simulink model "tcp_ip"  (R2021b)
settings: Solver=ode5  StartTime=0.0  StopTime=inf  FixedStep=1/20  RelTol=1e-3
PreLoadFcn:
  | mbxruntime.callbacks.PreLoadFcn(bdroot);
PostLoadFcn:
  | mbxruntime.callbacks.PostLoadFcn(bdroot);
InitFcn:
  | mbxruntime.callbacks.InitFcn(bdroot);
StartFcn:
  | mbxruntime.callbacks.StartFcn(bdroot);
StopFcn:
  | mbxruntime.callbacks.StopFcn(bdroot);
model workspace: external: MAT-File .\kea_demo_0218_cs_hws.mat (data not in the file)
undefined symbols (not defined in the file): DiscIntNeverNeededParam, kea_demo_0218_cs_1d5c9b61e8e009e5, kea_demo_0218_cs_4669f259e7287783, kea_demo_0218_cs_87ee11d7829c0052, kea_demo_0218_cs_Audi_A3_1_Dynamics_Simple_initialPitch, kea_demo_0218_cs_Audi_A3_1_Dynamics_Simple_initialRoll, kea_demo_0218_cs_Audi_A3_1_Dynamics_Simple_initialX, kea_demo_0218_cs_Audi_A3_1_Dynamics_Simple_initialY, kea_demo_0218_cs_Audi_A3_1_Dynamics_Simple_initialYaw, kea_demo_0218_cs_Audi_A3_1_Dynamics_Simple_initialZ, kea_demo_0218_cs_Audi_A3_1_PathFollower_Preview_1_PathUniqueID, kea_demo_0218_cs_Roewe_550_S_Sedan_1_Dynamics_Simple_initialX, kea_demo_0218_cs_Roewe_550_S_Sedan_1_Dynamics_Simple_initialY, kea_demo_0218_cs_Roewe_550_S_Sedan_1_Dynamics_Simple_initialYaw, kea_demo_0218_cs_Roewe_550_S_Sedan_1_Dynamics_Simple_initialZ, mbxruntime, warningInitialVelocity, x0
libraries: simulink x56, simulink_extras x18, instrumentlib x2
(part 4 of 7)

== system tcp_ip/Audi_A3_1/Dynamics_Simple/State2Bus1/state2FullState ==
  note: wrt GLOB
  note: Angles
      | wrtINI
  note: mode: Positioning
      | VelVEHICLE
      | wrt INI
  note: mode: Dynamics
      | VelVEHICLE
      | wrt VEH
  note: AnglesBODY
      | wrt GLOB
  note: AnglesVEHICLE
      | wrtGLOB
  note: AnglesBODY
      | wrtVEH
  dx,dy,dz [m/s] R,P,Y [rad] : Inport
  ini VEHpos wrt GLOB axis system [m] : Inport  Port=2
  iniBODY Angles wrt VEH axis system [deg] : Inport  Port=3
  iniVEH Angles wrt GLOB axis system [deg] : Inport  Port=4
  Degrees to Radians : simulink_extras/Transformations/Degrees to Radians
  Degrees to Radians1 : simulink_extras/Transformations/Degrees to Radians
  Demux : Demux  Outputs=3
  Demux1 : Demux  Outputs=[3 3 3]
  Demux2 : Demux  Outputs=[2 1]
  Demux3 : Demux  Outputs=2
  Demux4 : Demux  Outputs=3
  Discrete Derivative : simulink/Discrete/Discrete Derivative  gainval=1.0  ICPrevScaledInput=0.0  OutMin=[]  OutMax=[]  OutDataType=fixdt(1, 16)  OutScaling=2^-10  DoSatur=off
  Discrete Derivative1 : simulink/Discrete/Discrete Derivative  gainval=1.0  ICPrevScaledInput=0.0  OutMin=[]  OutMax=[]  OutDataType=fixdt(1, 16)  OutScaling=2^-10  DoSatur=off
  Discrete Derivative2 : simulink/Discrete/Discrete Derivative  gainval=1.0  ICPrevScaledInput=0.0  OutMin=[]  OutMax=[]  OutDataType=fixdt(1, 16)  OutScaling=2^-10  DoSatur=off
  Discrete Derivative3 : simulink/Discrete/Discrete Derivative  gainval=1.0  ICPrevScaledInput=str2num(get_param(gcb,'gainval'))*((Roll0*pi/180)/TimeStep)  OutMin=[]  OutMax=[]  OutDataType=fixdt(1, 16)  OutScaling=2^-10  DoSatur=off
  Discrete Derivative4 : simulink/Discrete/Discrete Derivative  gainval=1.0  ICPrevScaledInput=str2num(get_param(gcb,'gainval'))*((Pitch0*pi/180)/TimeStep)  OutMin=[]  OutMax=[]  OutDataType=fixdt(1, 16)  OutScaling=2^-10  DoSatur=off
  Discrete Derivative5 : simulink/Discrete/Discrete Derivative  gainval=1.0  ICPrevScaledInput=str2num(get_param(gcb,'gainval'))*((Yaw0*pi/180)/TimeStep)  OutMin=[]  OutMax=[]  OutDataType=fixdt(1, 16)  OutScaling=2^-10  DoSatur=off
  Mux : Mux  Inputs=[3 3 3 3 3]
  Mux1 : Mux  Inputs=3
  Mux2 : Mux  Inputs=3
  Sum : Sum  Inputs=|++
  Sum1 : Sum
  Sum2 : Sum
  Sum3 : Sum
  Transformation_BODY2GLOBAL : Subsystem
  Transformation_BODY2GLOBAL1 : Subsystem
  limit roll : Subsystem
  mux2 : Mux  Inputs=3
  mux3 : Mux  Inputs=3
  pitch_vehicle : Constant  Value=0
  roll_vehicle : Constant  Value=0
  yaw_body : Constant  Value=0
  State : Outport  VectorParamsAs1DForOutWhenUnconnected=off
  wires:
  Discrete Derivative5/1 -> Mux2/3
  Demux4/3 -> Discrete Derivative5/1
  Discrete Derivative4/1 -> Mux2/2
  Demux4/2 -> Discrete Derivative4/1
  Demux4/1 -> Discrete Derivative3/1
  Discrete Derivative3/1 -> Mux2/1
  Discrete Derivative2/1 -> Mux1/3
  Demux/3 -> Discrete Derivative2/1
  Discrete Derivative1/1 -> Mux1/2
  Demux/2 -> Discrete Derivative1/1
  Demux/1 -> Discrete Derivative/1
  Mux1/1 -> Mux/3  "AccVEH wrt  GLOB"
  Demux3/2 -> mux2/2  "pitch"
  ini VEHpos wrt GLOB axis system [m]/1 -> Sum3/2
  Degrees to Radians/1 -> Transformation_BODY2GLOBAL1/2(angles_BODYwrtGLOB_[rad]), Transformation_BODY2GLOBAL/2(angles_BODYwrtGLOB_[rad]), Sum2/2
  Degrees to Radians1/1 -> Sum1/2
  Demux3/1 -> mux2/1  "roll"
  Demux1/3 -> Demux2/1
  Demux2/1 -> Demux3/1
  Demux2/2 -> mux3/3  "yaw"
  Sum3/1 -> Mux/1  "PosVEH wrt  GLOB"
  Transformation_BODY2GLOBAL1/1(POSvector_GLOBAL_[m]) -> Sum3/1
  Sum1/1 -> Sum/1
  Demux1/1 -> Transformation_BODY2GLOBAL1/1(POSvector_BODY_[m])
  Transformation_BODY2GLOBAL/1(Vvector_GLOBAL_[m/s]) -> Demux/1, Mux/2  "VelVEH wrt  GLOB"
  dx,dy,dz [m/s] R,P,Y [rad]/1 -> Demux1/1
  Demux1/2 -> Transformation_BODY2GLOBAL/1(Vvector_BODY_[m/s])
  Sum2/1 -> Sum/2
  mux3/1 -> Sum2/1
  yaw_body/1 -> mux2/3  "yaw"
  mux2/1 -> Sum1/1
  pitch_vehicle/1 -> mux3/2  "pitch"
  roll_vehicle/1 -> mux3/1  "roll"
  Sum/1 -> limit roll/1(RPY)
  iniBODY Angles wrt VEH axis system [deg]/1 -> Degrees to Radians1/1
  iniVEH Angles wrt GLOB axis system [deg]/1 -> Degrees to Radians/1
  limit roll/1(RPYcor) -> Demux4/1, Mux/4  "AnglesBODY wrt  GLOB"
  Mux/1 -> State/1
  Mux2/1 -> Mux/5  "VelAnglesBODY wrt GLOB"
  Discrete Derivative/1 -> Mux1/1

== system tcp_ip/Audi_A3_1/Dynamics_Simple/Transmission/Torque_Converter ==
  note: <= 0
  note: > 0
  note: To compensate for no hydraulic connection when in neutral gear
  nEngine_[rpm] : Inport
  nTransmission_[rpm] : Inport  Port=2
  Gear nr : Inport  Port=3
  Compare To Constant : simulink/Logic and Bit Operations/Compare To Constant  relop=<=  const=1  OutDataTypeStr=uint8  ZeroCross=off
  Compare To Zero : simulink/Logic and Bit Operations/Compare To Zero  relop=~=  OutDataTypeStr=uint8  ZeroCross=off
  Constant : Constant  Value=1/50
  Constant1 : Constant
  Constant2 : Constant
  Drag : Gain  Gain=-1
  FactorK : Lookup  InputValues=p.speedratio  Table=p.Kfactor*p.Kcorr  SaturateOnIntegerOverflow=on
  Impeller : Fcn  Expr=u^2
  Product : Product  RndMeth=Zero
  Product1 : Product  RndMeth=Zero
  Quotient : Product  Inputs=*/  InputSameDT=on  SaturateOnIntegerOverflow=on  OutDataTypeStr=Inherit: Same as first input
  SpeedRatio : Product  Inputs=*/  InputSameDT=on  SaturateOnIntegerOverflow=on  OutDataTypeStr=Inherit: Same as first input
  Sum : Sum  Inputs=|+-
  Switch : Switch  Criteria=u2 ~= 0  Threshold=0.5
  Switch1 : Switch  Criteria=u2 ~= 0
  TorqueRatio : Lookup  InputValues=[p.speedratio 1]  Table=[p.Torqueratio 0]  SaturateOnIntegerOverflow=on
  Turbine : Product  InputSameDT=on  SaturateOnIntegerOverflow=on  OutDataTypeStr=Inherit: Same as first input
  rpm2rads-1 : Gain  Gain=2*pi/60
  ImpellerTorque_[Nm] : Outport  InitialOutput=0  VectorParamsAs1DForOutWhenUnconnected=off
  TurbineTorque_[Nm] : Outport  Port=2  InitialOutput=0  VectorParamsAs1DForOutWhenUnconnected=off
  wires:
  rpm2rads-1/1 -> Quotient/1
  Turbine/1 -> Switch1/1
  TorqueRatio/1 -> Turbine/2
  Compare To Constant/1 -> Switch1/2
  Constant2/1 -> Sum/2
  Sum/1 -> Drag/1
  Drag/1 -> Switch1/3
  Product1/1 -> TurbineTorque_[Nm]/1
  Switch1/1 -> Product1/2
  Compare To Zero/1 -> Switch/2
  Gear nr/1 -> Compare To Zero/1
  Constant1/1 -> Switch/1
  Constant/1 -> Switch/3
  Switch/1 -> Product1/1, Product/1
  Product/1 -> ImpellerTorque_[Nm]/1
  Quotient/1 -> Impeller/1
  FactorK/1 -> Quotient/2
  SpeedRatio/1 -> FactorK/1, Sum/1, Compare To Constant/1, TorqueRatio/1
  Impeller/1 -> Turbine/1, Product/2
  nEngine_[rpm]/1 -> SpeedRatio/2, rpm2rads-1/1
  nTransmission_[rpm]/1 -> SpeedRatio/1

== system tcp_ip/Audi_A3_1/Dynamics_Simple/Transmission/Transmission_Ratio ==
  tTransmissionIn_[Nm] : Inport
  GearNr_[-] : Inport  Port=2
  nTransmissionOut_[rpm] : Inport  Port=3
  Ensure positive TransmissionRPM : Abs
  If : If  IfExpression=u1 == 0  ElseIfExpressions=u1 == -1
  If Action Neutral : Subsystem  TreatAsAtomicUnit=on
  If Action Normal : Subsystem  TreatAsAtomicUnit=on
  If Action Reverse : Subsystem  TreatAsAtomicUnit=on
  Merge : Merge  Inputs=3
  OutputTorque = 0 : Constant  Value=0
  Product : Product  InputSameDT=on  SaturateOnIntegerOverflow=on  OutDataTypeStr=Inherit: Same as first input
  Product1 : Product  InputSameDT=on  SaturateOnIntegerOverflow=on  OutDataTypeStr=Inherit: Same as first input
  Transmission Gear ratios : Lookup  InputValues=p.tr_in  Table=p.tr_out  SaturateOnIntegerOverflow=on
  tTransmissionOut_[Nm] : Outport  InitialOutput=0  VectorParamsAs1DForOutWhenUnconnected=off
  nTransmissionIn_[rpm] : Outport  Port=2  InitialOutput=0  VectorParamsAs1DForOutWhenUnconnected=off
  wires:
  GearNr_[-]/1 -> Transmission Gear ratios/1, If/1
  If/3 -> If Action Normal/Action
  If/2 -> If Action Reverse/Action
  If Action Normal/1(Out1) -> Merge/3
  If Action Reverse/1(Out1) -> Merge/2
  If/1 -> If Action Neutral/Action
  If Action Neutral/1(Out1) -> Merge/1
  Product1/1 -> Ensure positive TransmissionRPM/1
  Merge/1 -> tTransmissionOut_[Nm]/1
  Product/1 -> If Action Reverse/1(In1), If Action Normal/1(In1)
  OutputTorque = 0/1 -> If Action Neutral/1(In1)
  Transmission Gear ratios/1 -> Product/2, Product1/1
  nTransmissionOut_[rpm]/1 -> Product1/2
  tTransmissionIn_[Nm]/1 -> Product/1
  Ensure positive TransmissionRPM/1 -> nTransmissionIn_[rpm]/1

== system tcp_ip/Audi_A3_1/PathFollower_Preview_1/LateralController/Calculate delta wheel ==
  In1 : Inport
  In2 : Inport  Port=2
  In3 : Inport  Port=3
  In4 : Inport  Port=4
  In5 : Inport  Port=5
  In6 : Inport  Port=6
  In7 : Inport  Port=7
  In8 : Inport  Port=8
  In9 : Inport  Port=9
  In10 : Inport  Port=10
  In11 : Inport  Port=11
  In12 : Inport  Port=12
  eml_delta_steering_error : MATLAB Function  TreatAsAtomicUnit=on  RTWFcnName=sfun_delta_steering_error  RTWFileName=sfun_delta_steering_error
      settings: RTWFileNameOpts=User specified
  Out1 : Outport  VectorParamsAs1DForOutWhenUnconnected=off
  wires:
  In3/1 -> eml_delta_steering_error/3(t_Preview_LatCtrl)
  In2/1 -> eml_delta_steering_error/2(v_x_vehicle_Min)
  In12/1 -> eml_delta_steering_error/12(wheelbase)
  In11/1 -> eml_delta_steering_error/11(Pos_x_CoG_Vehicle)
  In10/1 -> eml_delta_steering_error/10(e_Lat)
  In9/1 -> eml_delta_steering_error/9(inertia_z_vehicle_total)
  In8/1 -> eml_delta_steering_error/8(m_vehicle_total)
  eml_delta_steering_error/1(delta_steeringwheeltotal) -> Out1/1
  In7/1 -> eml_delta_steering_error/7(CorneringStiffness_Tyres_Rear)
  In6/1 -> eml_delta_steering_error/6(CorneringStiffness_Tyres_Front)
  In5/1 -> eml_delta_steering_error/5(yawrate_vehicle)
  In4/1 -> eml_delta_steering_error/4(v_y_vehicle)
  In1/1 -> eml_delta_steering_error/1(v_x_vehicle)

== system tcp_ip/Audi_A3_1/PathFollower_Preview_1/LateralController/SteeringWheelAngle ==
  Angle_Steering[rad] : Inport
  i_Steering[] : Inport  Port=2
  Angle_SteeringWheel_Last[deg] : Inport  Port=3
  LatCtrl1_Enable[0Off|1On] : Inport  Port=4
  Angle_Max_SteeringWheel[deg]1 : Constant  Value=Angle_Max_SteeringWheel  SampleTime=CSSampleTime
  Const_t_PT1_LatCtrl[s] : Constant  Value=DelayTime  SampleTime=CSSampleTime
  FirstOrderDynamics : Subsystem  mask(First Order Dynamics){}
      mask Display:
      | port_label('input',1,'In')
      | port_label('input',2,'T')
      | port_label('input',3,'Reset')
      | port_label('input',4,'x0')
      | 
      | plot([0.4 0.95], [0.1 0.1]);
      | plot([0.4 0.4], [0.1 0.95]);
      | plot(0.4 + 0.5*[0:0.1:1],0.8- 0.7 * exp(-5*[0:0.1:1]));
  Gain : Gain  SaturateOnIntegerOverflow=on  OutDataTypeStr=Inherit: Same as input  ParamDataTypeStr=Inherit: Same as input
  Product : Product  SaturateOnIntegerOverflow=on  OutDataTypeStr=Inherit: Same as first input
  Rate Limiter : RateLimiter  RisingSlewLimit=MaxSteeringRate  FallingSlewLimit=-MaxSteeringRate  SampleTimeMode=inherited
  Sat_Total : Subsystem
      mask Display:
      | plot([0.25 0.4 0.6 0.75],[0.2 0.2 0.8 0.8])
      | port_label('input',2,'Lim')
      | port_label('output',2,'Info')
  Terminator1 : Terminator
  rad2deg : Gain  Gain=180/pi  SaturateOnIntegerOverflow=on  OutDataTypeStr=Inherit: Same as input  ParamDataTypeStr=Inherit: Same as input
  Angle_SteeringWheel[deg] : Outport  VectorParamsAs1DForOutWhenUnconnected=off
  wires:
  Rate Limiter/1 -> FirstOrderDynamics/1(In)
  Gain/1 -> FirstOrderDynamics/3(Reset)
  Angle_SteeringWheel_Last[deg]/1 -> FirstOrderDynamics/4(x0)
  LatCtrl1_Enable[0Off|1On]/1 -> Gain/1
  Const_t_PT1_LatCtrl[s]/1 -> FirstOrderDynamics/2(TimeConstant[s])
  Sat_Total/2(Sat_Info) -> Terminator1/1
  Angle_Steering[rad]/1 -> rad2deg/1
  i_Steering[]/1 -> Product/2
  rad2deg/1 -> Product/1
  Product/1 -> Sat_Total/1(In)
  Sat_Total/1(Sat_Total) -> Rate Limiter/1
  FirstOrderDynamics/1(Out) -> Angle_SteeringWheel[deg]/1
  Angle_Max_SteeringWheel[deg]1/1 -> Sat_Total/2(Sat_Limit)

== system tcp_ip/Audi_A3_1/PathFollower_Preview_1/LateralController/s_Preview_LatCtrl ==
  v_x_Vehicle[m|s] : Inport
  v_x_Vehicle_Min[m|s] : Inport  Port=2
  t_Preview_LatCtrl[s] : Inport  Port=3
  Max : MinMax  Function=max  Inputs=2  InputSameDT=on  SaturateOnIntegerOverflow=on
  Prod_s_Min : Product  SaturateOnIntegerOverflow=on  OutDataTypeStr=Inherit: Same as first input
  Product : Product  SaturateOnIntegerOverflow=on  OutDataTypeStr=Inherit: Same as first input
  s_Preview_LatCtrl[m] : Outport  VectorParamsAs1DForOutWhenUnconnected=off
  wires:
  Max/1 -> s_Preview_LatCtrl[m]/1
  Prod_s_Min/1 -> Max/2
  v_x_Vehicle_Min[m|s]/1 -> Prod_s_Min/2
  t_Preview_LatCtrl[s]/1 -> Prod_s_Min/1, Product/2
  Product/1 -> Max/1
  v_x_Vehicle[m|s]/1 -> Product/1

== system tcp_ip/Audi_A3_1/PathFollower_Preview_1/LongitudinalController/Check_Initial_Velocity ==
  " v_actual_[m|s]" : Inport
  Initial_Velocity_[m|s] : Inport  Port=2
  > eps : simulink/Logic and Bit Operations/Compare To Constant  relop=>  const=0.1  OutDataTypeStr=boolean
  Abs : Abs
  Assertion : Assertion  AssertionFailFcn=warningInitialVelocity(PathFollowerBlockPath);  StopWhenAssertionFail=off
  Constant : Constant  Value=false
  First ? : Memory  InitialCondition=1
  Logical Operator : Logic  AllPortsSameDT=off  OutDataTypeStr=boolean
  Logical Operator1 : Logic  Operator=NOT  AllPortsSameDT=off  OutDataTypeStr=boolean
  Sum : Sum  Inputs=+-
  wires:
  Logical Operator1/1 -> Assertion/1
  Logical Operator/1 -> Logical Operator1/1
  Constant/1 -> First ?/1
  First ?/1 -> Logical Operator/2
  > eps/1 -> Logical Operator/1
  Sum/1 -> Abs/1
  Abs/1 -> > eps/1
  Initial_Velocity_[m|s]/1 -> Sum/2
  " v_actual_[m|s]"/1 -> Sum/1

== system tcp_ip/Audi_A3_1/PathFollower_Preview_1/LongitudinalController/If Desired Velocity = 0 ==
  In1 : Inport
  Action Port : ActionPort  InitializeStates=reset  PropagateVarSize=During execution  ActionPortLabel=if(u1 == 0)
  constant : Constant  Value=0
  constant1 : Constant  Value=150
  throttle [%] : Outport  InitialOutput=[0]  VectorParamsAs1DForOutWhenUnconnected=off
  brake pressure [bar] : Outport  Port=2  InitialOutput=[150]  VectorParamsAs1DForOutWhenUnconnected=off
  Auto_GearShift : Outport  Port=3  VectorParamsAs1DForOutWhenUnconnected=off
  wires:
  In1/1 -> Auto_GearShift/1
  constant/1 -> throttle [%]/1
  constant1/1 -> brake pressure [bar]/1

== system tcp_ip/Audi_A3_1/PathFollower_Preview_1/LongitudinalController/If Desired Velocity ~= 0 ==
  note: No brake/throttle actions
      | in case of small ctrl error,
      |  in order to prevent nervous
      | ctrl behaviour
  note: CONSTANT VELOCITY CONTROL
  In1 : Inport
  Desired Velocity [m/s] : Inport  Port=2
  Action Port : ActionPort  InitializeStates=reset  PropagateVarSize=During execution  ActionPortLabel=else
  Dead Zone1 : DeadZone  LowerValue=-10  UpperValue=1  SaturateOnIntegerOverflow=on
  Gain1 : Gain  Gain=-1
  Gain2 : Gain  Gain=1.5
  Limiter_brake : Saturate  UpperLimit=150  LowerLimit=0
  Limiter_throttle : Saturate  UpperLimit=100  LowerLimit=0
  PID_AWU : Subsystem  mask(PID Controller){P=LongCtrl_P, I=LongCtrl_I, D=LongCtrl_D}
      mask prompts: P "Proportional:"; I "Integral:"; D "Derivative:"
      mask help:
      | Enter expressions for proportional, integral, and derivative terms.
      | P+I/s+Ds
      mask Help: This block implements a PID controller where parameters are entered for the Proportional, Integral and Derivative terms. Unmask this block to see how it works. The derivative term is implemented using a true derivative block.
      mask Display: disp('PID')
  throttle [%] : Outport  VectorParamsAs1DForOutWhenUnconnected=off
  brake pressure [bar] : Outport  Port=2  VectorParamsAs1DForOutWhenUnconnected=off
  Auto_GearShift : Outport  Port=3  VectorParamsAs1DForOutWhenUnconnected=off
  wires:
  Dead Zone1/1 -> Gain2/1, Limiter_throttle/1
  Gain1/1 -> Limiter_brake/1
  Gain2/1 -> Gain1/1
  PID_AWU/1(u) -> Dead Zone1/1
  Desired Velocity [m/s]/1 -> PID_AWU/1(e)
  In1/1 -> Auto_GearShift/1
  Limiter_brake/1 -> brake pressure [bar]/1
  Limiter_throttle/1 -> throttle [%]/1  "throttle"

== system tcp_ip/Audi_A3_1/PathFollower_Preview_1/LongitudinalController/Memory External IC ==
  note: Xnew
  note: Initial Value
  u : Inport
  IC : Inport  Port=2
  FixPt Constant : Constant  DisableCoverage=on  Value=0  OutDataTypeStr=fixdt(0,8,0)
  FixPt Data Type Duplicate1 : DataTypeDuplicate  DisableCoverage=on  NumInputPorts=3
  Init : Switch  Criteria=u2 ~= 0  OutDataTypeStr=Inherit: Inherit via back propagation  ZeroCross=off
  Memory : Memory  InitialCondition=1  InheritSampleTime=on
  Memory1 : Memory  InheritSampleTime=on
  y : Outport  VectorParamsAs1DForOutWhenUnconnected=off
  wires:
  Memory1/1 -> Init/3  "Xold"
  Init/1 -> y/1, FixPt Data Type Duplicate1/1
  Memory/1 -> Init/2
  FixPt Constant/1 -> Memory/1
  u/1 -> Memory1/1, FixPt Data Type Duplicate1/2
  IC/1 -> Init/1, FixPt Data Type Duplicate1/3

== system tcp_ip/Audi_A3_1/SELF_Demux/compas converter/cart2compas ==
  Angle [deg] : Inport
  Constant : Constant  Value=90
  Constant1 : Constant  Value=360
  Gain : Gain  Gain=1/360
  Gain1 : Gain  Gain=360
  Gain2 : Gain  Gain=-1
  Rounding Function : Rounding
  Sum : Sum  Inputs=|-+
  Sum1 : Sum  Inputs=-+|
  Sum2 : Sum  Inputs=++|
  heading [deg] : Outport  VectorParamsAs1DForOutWhenUnconnected=off
  wires:
  Gain/1 -> Rounding Function/1
  Rounding Function/1 -> Gain1/1
  Gain1/1 -> Sum/1
  Angle [deg]/1 -> Sum1/2
  Sum/1 -> Gain2/1
  Sum1/1 -> Gain/1, Sum/2
  Constant/1 -> Sum1/1
  Gain2/1 -> Sum2/2
  Constant1/1 -> Sum2/1
  Sum2/1 -> heading [deg]/1

== system tcp_ip/Roewe_550_S_Sedan_1/Dynamics_Simple/Chassis/Bicycle_model_[XYZ] ==
  DeltaWheel_[rad] : Inport
  zFront_[m]_dzFront_[ms-1] : Inport  Port=2  PortDimensions=2
  zRear_[m]_dzRear_[ms-1] : Inport  Port=3  PortDimensions=2
  BrakePressure_[bar] : Inport  Port=4
  DriveTorque_[Nm] : Inport  Port=5
  v0_[ms-1] : Inport  Port=6
  |vx|_[ms-1] : Inport  Port=7
  Fy_rear_[N] : Inport  Port=8
  Fy_front_[N] : Inport  Port=9
  Demux : Demux  Outputs=2
  Demux1 : Demux  Outputs=2
  Fyi --> Fy / Mz : Subsystem
  X_Motion : Subsystem
  Y & Yaw_Motion : Subsystem
  "Z, Pitch_Motion & Roll_Motion" : Subsystem
  |vx|_[ms-1]1 : Outport  VectorParamsAs1DForOutWhenUnconnected=off
  vy_[ms-1] : Outport  Port=2  VectorParamsAs1DForOutWhenUnconnected=off
  vz_[ms-1] : Outport  Port=3  VectorParamsAs1DForOutWhenUnconnected=off
  RollAngle_[rad] : Outport  Port=4  VectorParamsAs1DForOutWhenUnconnected=off
  RollRate_[rads-1] : Outport  Port=5  VectorParamsAs1DForOutWhenUnconnected=off
  YawAngle_[rads-1] : Outport  Port=6  VectorParamsAs1DForOutWhenUnconnected=off
  Vx_[ms-1] : Outport  Port=7  VectorParamsAs1DForOutWhenUnconnected=off
  PitchAngle_[rad] : Outport  Port=8  VectorParamsAs1DForOutWhenUnconnected=off
  YawAngle_[rad] : Outport  Port=9  VectorParamsAs1DForOutWhenUnconnected=off
  ax_[ms-2] : Outport  Port=10  VectorParamsAs1DForOutWhenUnconnected=off
  ay_[ms-2] : Outport  Port=11  VectorParamsAs1DForOutWhenUnconnected=off
  wires:
  Fyi --> Fy / Mz/1(Fy_[N]) -> Y & Yaw_Motion/2(Fy_[N])  "Fy_[N]"
  Fyi --> Fy / Mz/2(Mz_[Nm]) -> Y & Yaw_Motion/3(Mz_[Nm])  "Mz_[Nm]"
  Y & Yaw_Motion/1(|vx|_[ms-1]1) -> |vx|_[ms-1]1/1  "|vx|_[ms-1]"
  Y & Yaw_Motion/2(vy_[ms-1]) -> vy_[ms-1]/1  "vy_[ms-1]"
  Y & Yaw_Motion/5(YawAngle_[rad]) -> YawAngle_[rad]/1  "YawAngle_[rad]"
  v0_[ms-1]/1 -> X_Motion/3(v0_[ms-1])  "v0_[ms-1]"
  BrakePressure_[bar]/1 -> X_Motion/2(BrakePressure_[bar])  "BrakePressure_[bar]"
  DriveTorque_[Nm]/1 -> X_Motion/1(DriveTorque_[Nm])  "DriveTorque_[Nm]"
  X_Motion/2(ax_[ms-2]) -> ax_[ms-2]/1, [ax]  "ax_[ms-2]"
  X_Motion/1(vx_[ms-1]) -> Vx_[ms-1]/1, [vx]  "vx_[ms-1]"
  [ax] -> "Z, Pitch_Motion & Roll_Motion"/3(ax)
  Demux/1 -> "Z, Pitch_Motion & Roll_Motion"/5(zFront_[m])
  Demux/2 -> "Z, Pitch_Motion & Roll_Motion"/6(dzFront_[ms-1])
  Demux1/1 -> "Z, Pitch_Motion & Roll_Motion"/7(zRear_[m])
  Demux1/2 -> "Z, Pitch_Motion & Roll_Motion"/8(dzRear_[ms-1])
  zRear_[m]_dzRear_[ms-1]/1 -> Demux1/1
  zFront_[m]_dzFront_[ms-1]/1 -> Demux/1
  "Z, Pitch_Motion & Roll_Motion"/2(vz_[ms-1]) -> vz_[ms-1]/1  "vz_[ms-1]"
  DeltaWheel_[rad]/1 -> Fyi --> Fy / Mz/1(DeltaWheel_[rad])
  Fy_front_[N]/1 -> Fyi --> Fy / Mz/2(Fy_f_[N])
  Fy_rear_[N]/1 -> Fyi --> Fy / Mz/3(Fy_r_[N])
  |vx|_[ms-1]/1 -> Y & Yaw_Motion/1(|vx|_[ms-1])
  Y & Yaw_Motion/3(ay_[ms-2]) -> [ay], ay_[ms-2]/1  "ay_[ms-2]"
  [ay] -> "Z, Pitch_Motion & Roll_Motion"/4(ay)
  "Z, Pitch_Motion & Roll_Motion"/3(RollAngle_[rad]) -> RollAngle_[rad]/1  "RollAngle_[rad]"
  "Z, Pitch_Motion & Roll_Motion"/4(RollRate_[rads-1]) -> RollRate_[rads-1]/1  "RollRate_[rads-1]"
  [dYaw] -> "Z, Pitch_Motion & Roll_Motion"/2(dYaw)
  [vx] -> "Z, Pitch_Motion & Roll_Motion"/1(vx)
  Y & Yaw_Motion/4(dYawAngle_[rads-1]) -> YawAngle_[rads-1]/1, [dYaw]  "dYawAngle_[rads-1]"
  "Z, Pitch_Motion & Roll_Motion"/1(pitchAngle_[rad]) -> PitchAngle_[rad]/1  "PitchAngle_[rad]"

== system tcp_ip/Roewe_550_S_Sedan_1/Dynamics_Simple/Chassis/FrontTyre ==
  note: alpha limiter
      | [-1 ... 1]
  note: relax_on
      | ON: 1
      | OFF: 0
  note: MOTORCYCLE ONLY
  note: VEHICLE + MOTORCYCLE
  DeltaWheel_[rad] : Inport
  |vx|_[ms-1] : Inport  Port=2
  vy_[ms-1] : Inport  Port=3
  dYawAngle_[rads-1] : Inport  Port=4
  RollAngle_[rad] : Inport  Port=5
  AlphaFront : Subsystem
  Compare To Zero : simulink/Logic and Bit Operations/Compare To Zero  relop===  OutDataTypeStr=boolean  ZeroCross=off
  Configurable Subsystem : Subsystem  Variant=on  VariantControlMode=label  LabelModeActiveChoice=Continuous
      settings: AttributesFormatString=%<BlockChoice>  OpenFcn=BringToFront(gcb);
  Configurable Subsystem1 : Subsystem  Variant=on  VariantControlMode=label  LabelModeActiveChoice=Continuous
      settings: AttributesFormatString=%<BlockChoice>  OpenFcn=BringToFront(gcb);
  Constant : Constant  Value=p.relax_on
  Constant1 : Constant  Value=p.relax_on
  Constant2 : Constant  Value=p.VehMCSwitch
  Data Type Conversion : DataTypeConversion  OutDataTypeStr=double
  If MC : simulink/Logic and Bit Operations/Compare To Constant  relop===  const=2  OutDataTypeStr=uint8  ZeroCross=off
  K_gamma_front : Gain  Gain=p.Kgfront
  Linl : Fcn  Expr=(u(4) - u(5))/p.sigma_front*u(1)
  Linl1 : Fcn  Expr=(u(4) - u(5))/p.sigma_front*u(1)
  Mux1 : Mux  Inputs=3
  Mux2 : Mux  Inputs={3,1,1}
  Mux3 : Mux  Inputs={3,1,1}
  Prevent_instability_at_low_Vx : Subsystem
  Product : Product  RndMeth=Zero
  Sum : Sum  Inputs=|++  InputSameDT=on  SaturateOnIntegerOverflow=on  OutDataTypeStr=Inherit: Same as first input
  Sum1 : Sum  Inputs=|++
  Switch : Switch  Threshold=0.5  SaturateOnIntegerOverflow=on  InputSameDT=on
  Switch1 : Switch  Threshold=0.5  SaturateOnIntegerOverflow=on  InputSameDT=on
  alg.loop : Memory
  due to sign convention : Gain  Gain=-1  SaturateOnIntegerOverflow=on  OutDataTypeStr=Inherit: Same as input  ParamDataTypeStr=Inherit: Same as input
  front_tyre : Gain  Gain=p.Kfront
  FyFront_[N] : Outport  VectorParamsAs1DForOutWhenUnconnected=off
  wires:
  Prevent_instability_at_low_Vx/1(alpha [rad]) -> Mux2/2, Switch/3
  Sum/1 -> Prevent_instability_at_low_Vx/1(alpha[rad])  "AlphaStatFront_[rad]"
  Switch/1 -> front_tyre/1  "AlphaFront_[rad]"
  Constant/1 -> Switch/2
  Sum1/1 -> FyFront_[N]/1  "FyFront_[N]"
  Mux2/1 -> Linl/1
  Linl/1 -> Configurable Subsystem/1(In1)
  Configurable Subsystem/1(Out1) -> Mux2/3, Switch/1  "AlphaRelaxFront_[rad]"
  AlphaFront/1(Alpha) -> Sum/1
  Mux1/1 -> Prevent_instability_at_low_Vx/2(In), AlphaFront/1(In), Mux2/1, Mux3/1
  |vx|_[ms-1]/1 -> Mux1/1, Compare To Zero/1
  vy_[ms-1]/1 -> Mux1/2
  dYawAngle_[rads-1]/1 -> Mux1/3
  alg.loop/1 -> Switch1/3
  Configurable Subsystem1/1(Out1) -> Mux3/3, Switch1/1  "GammaRelaxFront_[rad]"
  Linl1/1 -> Configurable Subsystem1/1(In1)
  Mux3/1 -> Linl1/1
  Constant1/1 -> Switch1/2
  due to sign convention/1 -> alg.loop/1, Mux3/2  "GammaStatFront_[rad]"
  RollAngle_[rad]/1 -> due to sign convention/1
  front_tyre/1 -> Sum1/1
  Constant2/1 -> If MC/1
  If MC/1 -> Data Type Conversion/1
  K_gamma_front/1 -> Product/1
  Product/1 -> Sum1/2
  Data Type Conversion/1 -> Product/2
  Compare To Zero/1 -> [reset]
  [reset] -> Configurable Subsystem/2(In2)
  [reset] -> Configurable Subsystem1/2(In2)
  DeltaWheel_[rad]/1 -> Sum/2  "DeltaWheel_[rad]"
  Switch1/1 -> K_gamma_front/1  "GammaFront_[rad]"

== system tcp_ip/Roewe_550_S_Sedan_1/Dynamics_Simple/Chassis/MuxDynState ==
  note: The position inputs are computed by the
      | integrated velocity.
  note: mode: Dynamics
      | VelVEHICLE
      | wrt VEH
  note: AnglesVEHICLE
      | wrtGLOB
  vx [ms-1] : Inport
  vy [ms-1] : Inport  Port=2
  vz [ms-1] : Inport  Port=3
  R [rad] : Inport  Port=4
  P [rad] : Inport  Port=5
  Y [rad] : Inport  Port=6
  Configurable Subsystem1 : Subsystem  Variant=on  VariantControlMode=label  LabelModeActiveChoice=Continuous  mask{IntegrationMethod=Integrator: Forward Euler}
      mask prompts: IntegrationMethod "Integration method"
      mask init: same as tcp_ip/Audi_A3_1/Dynamics_Simple/Chassis/MuxDynState/Configurable Subsystem1
      settings: AttributesFormatString=%<BlockChoice>  OpenFcn=BringToFront(gcb);
      mask TypeOptions IntegrationMethod: Integrator: Forward Euler | Integrator: Backward Euler
  Ground : Ground
  Ground1 : Ground
  Mux : Mux  Inputs=[3 3 3]
  Mux1 : Mux  Inputs=3
  Mux2 : Mux  Inputs=3
  Transformation_BODY2GLOBAL : Subsystem
  mux3 : Mux  Inputs=3
  State : Outport  VectorParamsAs1DForOutWhenUnconnected=off
  wires:
  Ground1/1 -> mux3/2  "pitch"
  Y [rad]/1 -> Mux2/3, mux3/3  "yaw"
  P [rad]/1 -> Mux2/2
  R [rad]/1 -> Mux2/1
  vz [ms-1]/1 -> Mux1/3
  vy [ms-1]/1 -> Mux1/2
  vx [ms-1]/1 -> Mux1/1
  Mux2/1 -> Mux/3
  Transformation_BODY2GLOBAL/1(Vvector_GLOBAL_[m/s]) -> Configurable Subsystem1/1(In1), Mux/2  "VelVEH wrt  GLOB"
  mux3/1 -> Transformation_BODY2GLOBAL/2(angles_BODYwrtGLOB_[rad])
  Ground/1 -> mux3/1  "roll"
  Mux/1 -> State/1
  Mux1/1 -> Transformation_BODY2GLOBAL/1(Vvector_BODY_[m/s])
  Configurable Subsystem1/1(Out1) -> Mux/1  "PosVEH wrt  GLOB"

== system tcp_ip/Roewe_550_S_Sedan_1/Dynamics_Simple/Chassis/Power Assisted Steering ==
  note: MOTORCYCLE
  note: VEHICLE
  note: Reverse steering direction for negative velocities
  Vx_[ms-1] : Inport
  Delta_in_[deg] : Inport  Port=2
  Constant : Constant
  Constant1 : Constant  Value=p.VehMCSwitch
  Lookup Table : Lookup  InputValues=[0 35 45 100]  Table=[1 1 0.2 0.2]
  Multiport Switch : MultiPortSwitch  Inputs=2
  Product : Product  Inputs=3  RndMeth=Zero
  Sign : Signum
  Delta_out_[deg] : Outport  VectorParamsAs1DForOutWhenUnconnected=off
  wires:
  Vx_[ms-1]/1 -> Lookup Table/1, Sign/1
  Delta_in_[deg]/1 -> Product/3
  Constant1/1 -> Multiport Switch/1
  Constant/1 -> Multiport Switch/3
  Lookup Table/1 -> Multiport Switch/2
  Multiport Switch/1 -> Product/2
  Product/1 -> Delta_out_[deg]/1
  Sign/1 -> Product/1

== system tcp_ip/Roewe_550_S_Sedan_1/Dynamics_Simple/Chassis/RearTyre ==
  note: alpha limiter
      | [-1 ... 1]
  note: relax_on
      | ON: 1
      | OFF: 0
  note: MOTORCYCLE ONLY
  note: VEHICLE + MOTORCYCLE
  |vx|_[ms-1] : Inport
  vy_[ms-1] : Inport  Port=2
  dpsi_[rads-1] : Inport  Port=3
  RollAngle_[rad] : Inport  Port=4
  AlphaRear : Subsystem
  Compare To Zero : simulink/Logic and Bit Operations/Compare To Zero  relop===  OutDataTypeStr=boolean  ZeroCross=off
  Configurable Subsystem : Subsystem  Variant=on  VariantControlMode=label  LabelModeActiveChoice=Continuous
      settings: AttributesFormatString=%<BlockChoice>  OpenFcn=BringToFront(gcb);
  Configurable Subsystem1 : Subsystem  Variant=on  VariantControlMode=label  LabelModeActiveChoice=Continuous
      settings: AttributesFormatString=%<BlockChoice>  OpenFcn=BringToFront(gcb);
  Constant1 : Constant  Value=p.relax_on
  Constant2 : Constant  Value=p.relax_on
  Constant3 : Constant  Value=p.VehMCSwitch
  Data Type Conversion : DataTypeConversion  OutDataTypeStr=double
  If MC : simulink/Logic and Bit Operations/Compare To Constant  relop===  const=2  OutDataTypeStr=uint8  ZeroCross=off
  K_gamma_rear : Gain  Gain=p.Kgrear
  Linl : Fcn  Expr=(u(4) - u(5))/p.sigma_rear*u(1)
  Linl1 : Fcn  Expr=(u(4) - u(5))/p.sigma_rear*u(1)
  Mux1 : Mux  Inputs=3
  Mux2 : Mux  Inputs={3,1,1}
  Mux3 : Mux  Inputs={3,1,1}
  Prevent_instability_at_low_Vx : Subsystem
  Product : Product  RndMeth=Zero
  Sum1 : Sum  Inputs=|++
  Switch1 : Switch  Threshold=0.5  SaturateOnIntegerOverflow=on  InputSameDT=on
  Switch2 : Switch  Threshold=0.5  SaturateOnIntegerOverflow=on  InputSameDT=on
  alg.loop : Memory
  due to sign convention : Gain  Gain=-1  SaturateOnIntegerOverflow=on  OutDataTypeStr=Inherit: Same as input  ParamDataTypeStr=Inherit: Same as input
  rear_tyre : Gain  Gain=p.Krear
  FyRear_[N] : Outport  VectorParamsAs1DForOutWhenUnconnected=off
  wires:
  Prevent_instability_at_low_Vx/1(alpha [rad]) -> Switch1/3, Mux2/2
  AlphaRear/1(Alpha) -> Prevent_instability_at_low_Vx/1(alpha[rad])  "AlphaStatRear_[rad]"
  Switch1/1 -> rear_tyre/1  "AlphaRear_[rad]"
  Constant1/1 -> Switch1/2
  Sum1/1 -> FyRear_[N]/1  "FyRear_[N]"
  Mux2/1 -> Linl/1
  Linl/1 -> Configurable Subsystem1/1(In1)
  Configurable Subsystem1/1(Out1) -> Mux2/3, Switch1/1  "AlphaRelaxRear_[rad]"
  Mux1/1 -> Prevent_instability_at_low_Vx/2(In), AlphaRear/1(In), Mux2/1, Mux3/1
  |vx|_[ms-1]/1 -> Mux1/1, Compare To Zero/1
  vy_[ms-1]/1 -> Mux1/2
  dpsi_[rads-1]/1 -> Mux1/3
  alg.loop/1 -> Switch2/3
  Configurable Subsystem/1(Out1) -> Mux3/3, Switch2/1  "GammaRelaxRear_[rad]"
  Linl1/1 -> Configurable Subsystem/1(In1)
  Mux3/1 -> Linl1/1
  Constant2/1 -> Switch2/2
  due to sign convention/1 -> alg.loop/1, Mux3/2  "GammaStatRear_[rad]"
  RollAngle_[rad]/1 -> due to sign convention/1
  Constant3/1 -> If MC/1
  If MC/1 -> Data Type Conversion/1
  Product/1 -> Sum1/2
  Data Type Conversion/1 -> Product/2
  K_gamma_rear/1 -> Product/1
  rear_tyre/1 -> Sum1/1
  Compare To Zero/1 -> [reset]
  [reset] -> Configurable Subsystem1/2(In2)
  [reset] -> Configurable Subsystem/2(In2)
  Switch2/1 -> K_gamma_rear/1  "GammaFront_[rad]"

== system tcp_ip/Roewe_550_S_Sedan_1/Dynamics_Simple/Engine/Configurable Subsystem ==
  In1 : Inport
  Discrete Rate Limiter : Subsystem  VariantControl=Discrete
  Rate Limiter : Subsystem  VariantControl=Continuous
  Out1 : Outport  VectorParamsAs1DForOutWhenUnconnected=off

== system tcp_ip/Roewe_550_S_Sedan_1/Dynamics_Simple/Engine/Configurable Subsystem1 ==
  In1 : Inport
  Discrete-Time Integrator : Subsystem  VariantControl=Discrete
  Integrator : Subsystem  VariantControl=Continuous
  Out1 : Outport  VectorParamsAs1DForOutWhenUnconnected=off

== system tcp_ip/Roewe_550_S_Sedan_1/Dynamics_Simple/Gear: Auto Manual/If Action Subsystem ==
  In1 : Inport
  Action Port : ActionPort  PropagateVarSize=During execution  ActionPortLabel=if(u1 == 0)
  Out1 : Outport  VectorParamsAs1DForOutWhenUnconnected=off
  wires:
  In1/1 -> Out1/1

== system tcp_ip/Roewe_550_S_Sedan_1/Dynamics_Simple/Gear: Auto Manual/If Action Subsystem1 ==
  In1 : Inport
  Action Port : ActionPort  PropagateVarSize=During execution  ActionPortLabel=else
  Out1 : Outport  VectorParamsAs1DForOutWhenUnconnected=off
  wires:
  In1/1 -> Out1/1

== system tcp_ip/Roewe_550_S_Sedan_1/Dynamics_Simple/ShiftLogic/Detect Increase ==
  GearNr_[-] : Inport
  In2 : Inport  Port=2
  Constant : Constant
  Data Type Conversion : DataTypeConversion  OutDataTypeStr=double
  Data Type Conversion1 : DataTypeConversion  OutDataTypeStr=double
  Detect Increase : simulink/Logic and Bit Operations/Detect Increase  vinit=1  OutDataTypeStr=uint8
  If : If  NumInputs=2  IfExpression="u1==1 &  u2==1"
  If V0 higher of the from 2->3 shifting velocity : Subsystem  TreatAsAtomicUnit=on
  Merge : Merge
  Other : Subsystem  TreatAsAtomicUnit=on
  Out1 : Outport  VectorParamsAs1DForOutWhenUnconnected=off
  wires:
  If/2 -> Other/Action
  If V0 higher of the from 2->3 shifting velocity/1(Out1) -> Merge/1
  Other/1(Out1) -> Merge/2
  Detect Increase/1 -> Data Type Conversion/1
  Merge/1 -> Out1/1
  If/1 -> If V0 higher of the from 2->3 shifting velocity/Action
  Data Type Conversion1/1 -> If/2
  Data Type Conversion/1 -> If/1
  Constant/1 -> If V0 higher of the from 2->3 shifting velocity/1(In1)
  GearNr_[-]/1 -> Detect Increase/1
  In2/1 -> Data Type Conversion1/1, Other/1(In1)

== system tcp_ip/Roewe_550_S_Sedan_1/Dynamics_Simple/ShiftLogic/If Action Neutral ==
  In1 : Inport
  Action Port : ActionPort  InitializeStates=reset  PropagateVarSize=During execution  ActionPortLabel=if(u1 == 0)
  Out1 : Outport  VectorParamsAs1DForOutWhenUnconnected=off
  wires:
  In1/1 -> Out1/1

== system tcp_ip/Roewe_550_S_Sedan_1/Dynamics_Simple/ShiftLogic/If Action Normal ==
  In1 : Inport
  Action Port : ActionPort  InitializeStates=reset  PropagateVarSize=During execution  ActionPortLabel=else
  Out1 : Outport  VectorParamsAs1DForOutWhenUnconnected=off
  wires:
  In1/1 -> Out1/1

== system tcp_ip/Roewe_550_S_Sedan_1/Dynamics_Simple/ShiftLogic/If Action Reverse ==
  In1 : Inport
  Action Port : ActionPort  InitializeStates=reset  PropagateVarSize=During execution  ActionPortLabel=elseif(u1 < 0)
  Out1 : Outport  VectorParamsAs1DForOutWhenUnconnected=off
  wires:
  In1/1 -> Out1/1

== system tcp_ip/Roewe_550_S_Sedan_1/Dynamics_Simple/State2Bus1/state2FullState ==
  note: wrt GLOB
  note: Angles
      | wrtINI
  note: mode: Positioning
      | VelVEHICLE
      | wrt INI
  note: mode: Dynamics
      | VelVEHICLE
      | wrt VEH
  note: AnglesBODY
      | wrt GLOB
  note: AnglesVEHICLE
      | wrtGLOB
  note: AnglesBODY
      | wrtVEH
  dx,dy,dz [m/s] R,P,Y [rad] : Inport
  ini VEHpos wrt GLOB axis system [m] : Inport  Port=2
  iniBODY Angles wrt VEH axis system [deg] : Inport  Port=3
  iniVEH Angles wrt GLOB axis system [deg] : Inport  Port=4
  Degrees to Radians : simulink_extras/Transformations/Degrees to Radians
  Degrees to Radians1 : simulink_extras/Transformations/Degrees to Radians
  Demux : Demux  Outputs=3
  Demux1 : Demux  Outputs=[3 3 3]
  Demux2 : Demux  Outputs=[2 1]
  Demux3 : Demux  Outputs=2
  Demux4 : Demux  Outputs=3
  Discrete Derivative : simulink/Discrete/Discrete Derivative  gainval=1.0  ICPrevScaledInput=0.0  OutMin=[]  OutMax=[]  OutDataType=fixdt(1, 16)  OutScaling=2^-10  DoSatur=off
  Discrete Derivative1 : simulink/Discrete/Discrete Derivative  gainval=1.0  ICPrevScaledInput=0.0  OutMin=[]  OutMax=[]  OutDataType=fixdt(1, 16)  OutScaling=2^-10  DoSatur=off
  Discrete Derivative2 : simulink/Discrete/Discrete Derivative  gainval=1.0  ICPrevScaledInput=0.0  OutMin=[]  OutMax=[]  OutDataType=fixdt(1, 16)  OutScaling=2^-10  DoSatur=off
  Discrete Derivative3 : simulink/Discrete/Discrete Derivative  gainval=1.0  ICPrevScaledInput=str2num(get_param(gcb,'gainval'))*((Roll0*pi/180)/TimeStep)  OutMin=[]  OutMax=[]  OutDataType=fixdt(1, 16)  OutScaling=2^-10  DoSatur=off
  Discrete Derivative4 : simulink/Discrete/Discrete Derivative  gainval=1.0  ICPrevScaledInput=str2num(get_param(gcb,'gainval'))*((Pitch0*pi/180)/TimeStep)  OutMin=[]  OutMax=[]  OutDataType=fixdt(1, 16)  OutScaling=2^-10  DoSatur=off
  Discrete Derivative5 : simulink/Discrete/Discrete Derivative  gainval=1.0  ICPrevScaledInput=str2num(get_param(gcb,'gainval'))*((Yaw0*pi/180)/TimeStep)  OutMin=[]  OutMax=[]  OutDataType=fixdt(1, 16)  OutScaling=2^-10  DoSatur=off
  Mux : Mux  Inputs=[3 3 3 3 3]
  Mux1 : Mux  Inputs=3
  Mux2 : Mux  Inputs=3
  Sum : Sum  Inputs=|++
  Sum1 : Sum
  Sum2 : Sum
  Sum3 : Sum
  Transformation_BODY2GLOBAL : Subsystem
  Transformation_BODY2GLOBAL1 : Subsystem
  limit roll : Subsystem
  mux2 : Mux  Inputs=3
  mux3 : Mux  Inputs=3
  pitch_vehicle : Constant  Value=0
  roll_vehicle : Constant  Value=0
  yaw_body : Constant  Value=0
  State : Outport  VectorParamsAs1DForOutWhenUnconnected=off
  wires:
  Discrete Derivative5/1 -> Mux2/3
  Demux4/3 -> Discrete Derivative5/1
  Discrete Derivative4/1 -> Mux2/2
  Demux4/2 -> Discrete Derivative4/1
  Demux4/1 -> Discrete Derivative3/1
  Discrete Derivative3/1 -> Mux2/1
  Discrete Derivative2/1 -> Mux1/3
  Demux/3 -> Discrete Derivative2/1
  Discrete Derivative1/1 -> Mux1/2
  Demux/2 -> Discrete Derivative1/1
  Demux/1 -> Discrete Derivative/1
  Mux1/1 -> Mux/3  "AccVEH wrt  GLOB"
  Demux3/2 -> mux2/2  "pitch"
  ini VEHpos wrt GLOB axis system [m]/1 -> Sum3/2
  Degrees to Radians/1 -> Transformation_BODY2GLOBAL1/2(angles_BODYwrtGLOB_[rad]), Transformation_BODY2GLOBAL/2(angles_BODYwrtGLOB_[rad]), Sum2/2
  Degrees to Radians1/1 -> Sum1/2
  Demux3/1 -> mux2/1  "roll"
  Demux1/3 -> Demux2/1
  Demux2/1 -> Demux3/1
  Demux2/2 -> mux3/3  "yaw"
  Sum3/1 -> Mux/1  "PosVEH wrt  GLOB"
  Transformation_BODY2GLOBAL1/1(POSvector_GLOBAL_[m]) -> Sum3/1
  Sum1/1 -> Sum/1
  Demux1/1 -> Transformation_BODY2GLOBAL1/1(POSvector_BODY_[m])
  Transformation_BODY2GLOBAL/1(Vvector_GLOBAL_[m/s]) -> Demux/1, Mux/2  "VelVEH wrt  GLOB"
  dx,dy,dz [m/s] R,P,Y [rad]/1 -> Demux1/1
  Demux1/2 -> Transformation_BODY2GLOBAL/1(Vvector_BODY_[m/s])
  Sum2/1 -> Sum/2
  mux3/1 -> Sum2/1
  yaw_body/1 -> mux2/3  "yaw"
  mux2/1 -> Sum1/1
  pitch_vehicle/1 -> mux3/2  "pitch"
  roll_vehicle/1 -> mux3/1  "roll"
  Sum/1 -> limit roll/1(RPY)
  iniBODY Angles wrt VEH axis system [deg]/1 -> Degrees to Radians1/1
  iniVEH Angles wrt GLOB axis system [deg]/1 -> Degrees to Radians/1
  limit roll/1(RPYcor) -> Demux4/1, Mux/4  "AnglesBODY wrt  GLOB"
  Mux/1 -> State/1
  Mux2/1 -> Mux/5  "VelAnglesBODY wrt GLOB"
  Discrete Derivative/1 -> Mux1/1

== system tcp_ip/Roewe_550_S_Sedan_1/Dynamics_Simple/Transmission/Torque_Converter ==
  note: <= 0
  note: > 0
  note: To compensate for no hydraulic connection when in neutral gear
  nEngine_[rpm] : Inport
  nTransmission_[rpm] : Inport  Port=2
  Gear nr : Inport  Port=3
  Compare To Constant : simulink/Logic and Bit Operations/Compare To Constant  relop=<=  const=1  OutDataTypeStr=uint8  ZeroCross=off
  Compare To Zero : simulink/Logic and Bit Operations/Compare To Zero  relop=~=  OutDataTypeStr=uint8  ZeroCross=off
  Constant : Constant  Value=1/50
  Constant1 : Constant
  Constant2 : Constant
  Drag : Gain  Gain=-1
  FactorK : Lookup  InputValues=p.speedratio  Table=p.Kfactor*p.Kcorr  SaturateOnIntegerOverflow=on
  Impeller : Fcn  Expr=u^2
  Product : Product  RndMeth=Zero
  Product1 : Product  RndMeth=Zero
  Quotient : Product  Inputs=*/  InputSameDT=on  SaturateOnIntegerOverflow=on  OutDataTypeStr=Inherit: Same as first input
  SpeedRatio : Product  Inputs=*/  InputSameDT=on  SaturateOnIntegerOverflow=on  OutDataTypeStr=Inherit: Same as first input
  Sum : Sum  Inputs=|+-
  Switch : Switch  Criteria=u2 ~= 0  Threshold=0.5
  Switch1 : Switch  Criteria=u2 ~= 0
  TorqueRatio : Lookup  InputValues=[p.speedratio 1]  Table=[p.Torqueratio 0]  SaturateOnIntegerOverflow=on
  Turbine : Product  InputSameDT=on  SaturateOnIntegerOverflow=on  OutDataTypeStr=Inherit: Same as first input
  rpm2rads-1 : Gain  Gain=2*pi/60
  ImpellerTorque_[Nm] : Outport  InitialOutput=0  VectorParamsAs1DForOutWhenUnconnected=off
  TurbineTorque_[Nm] : Outport  Port=2  InitialOutput=0  VectorParamsAs1DForOutWhenUnconnected=off
  wires:
  rpm2rads-1/1 -> Quotient/1
  Turbine/1 -> Switch1/1
  TorqueRatio/1 -> Turbine/2
  Compare To Constant/1 -> Switch1/2
  Constant2/1 -> Sum/2
  Sum/1 -> Drag/1
  Drag/1 -> Switch1/3
  Product1/1 -> TurbineTorque_[Nm]/1
  Switch1/1 -> Product1/2
  Compare To Zero/1 -> Switch/2
  Gear nr/1 -> Compare To Zero/1
  Constant1/1 -> Switch/1
  Constant/1 -> Switch/3
  Switch/1 -> Product1/1, Product/1
  Product/1 -> ImpellerTorque_[Nm]/1
  Quotient/1 -> Impeller/1
  FactorK/1 -> Quotient/2
  SpeedRatio/1 -> FactorK/1, Sum/1, Compare To Constant/1, TorqueRatio/1
  Impeller/1 -> Turbine/1, Product/2
  nEngine_[rpm]/1 -> SpeedRatio/2, rpm2rads-1/1
  nTransmission_[rpm]/1 -> SpeedRatio/1

== system tcp_ip/Roewe_550_S_Sedan_1/Dynamics_Simple/Transmission/Transmission_Ratio ==
  tTransmissionIn_[Nm] : Inport
  GearNr_[-] : Inport  Port=2
  nTransmissionOut_[rpm] : Inport  Port=3
  Ensure positive TransmissionRPM : Abs
  If : If  IfExpression=u1 == 0  ElseIfExpressions=u1 == -1
  If Action Neutral : Subsystem  TreatAsAtomicUnit=on
  If Action Normal : Subsystem  TreatAsAtomicUnit=on
  If Action Reverse : Subsystem  TreatAsAtomicUnit=on
  Merge : Merge  Inputs=3
  OutputTorque = 0 : Constant  Value=0
  Product : Product  InputSameDT=on  SaturateOnIntegerOverflow=on  OutDataTypeStr=Inherit: Same as first input
  Product1 : Product  InputSameDT=on  SaturateOnIntegerOverflow=on  OutDataTypeStr=Inherit: Same as first input
  Transmission Gear ratios : Lookup  InputValues=p.tr_in  Table=p.tr_out  SaturateOnIntegerOverflow=on
  tTransmissionOut_[Nm] : Outport  InitialOutput=0  VectorParamsAs1DForOutWhenUnconnected=off
  nTransmissionIn_[rpm] : Outport  Port=2  InitialOutput=0  VectorParamsAs1DForOutWhenUnconnected=off
  wires:
  GearNr_[-]/1 -> Transmission Gear ratios/1, If/1
  If/3 -> If Action Normal/Action
  If/2 -> If Action Reverse/Action
  If Action Normal/1(Out1) -> Merge/3
  If Action Reverse/1(Out1) -> Merge/2
  If/1 -> If Action Neutral/Action
  If Action Neutral/1(Out1) -> Merge/1
  Product1/1 -> Ensure positive TransmissionRPM/1
  Merge/1 -> tTransmissionOut_[Nm]/1
  Product/1 -> If Action Reverse/1(In1), If Action Normal/1(In1)
  OutputTorque = 0/1 -> If Action Neutral/1(In1)
  Transmission Gear ratios/1 -> Product/2, Product1/1
  nTransmissionOut_[rpm]/1 -> Product1/2
  tTransmissionIn_[Nm]/1 -> Product/1
  Ensure positive TransmissionRPM/1 -> nTransmissionIn_[rpm]/1

== system tcp_ip/Roewe_550_S_Sedan_1/PathFollower_Preview_1/LateralController/Calculate delta wheel ==
  In1 : Inport
  In2 : Inport  Port=2
  In3 : Inport  Port=3
  In4 : Inport  Port=4
  In5 : Inport  Port=5
  In6 : Inport  Port=6
  In7 : Inport  Port=7
  In8 : Inport  Port=8
  In9 : Inport  Port=9
  In10 : Inport  Port=10
  In11 : Inport  Port=11
  In12 : Inport  Port=12
  eml_delta_steering_error : MATLAB Function  TreatAsAtomicUnit=on  RTWFcnName=sfun_delta_steering_error  RTWFileName=sfun_delta_steering_error
      settings: RTWFileNameOpts=User specified
  Out1 : Outport  VectorParamsAs1DForOutWhenUnconnected=off
  wires:
  In3/1 -> eml_delta_steering_error/3(t_Preview_LatCtrl)
  In2/1 -> eml_delta_steering_error/2(v_x_vehicle_Min)
  In12/1 -> eml_delta_steering_error/12(wheelbase)
  In11/1 -> eml_delta_steering_error/11(Pos_x_CoG_Vehicle)
  In10/1 -> eml_delta_steering_error/10(e_Lat)
  In9/1 -> eml_delta_steering_error/9(inertia_z_vehicle_total)
  In8/1 -> eml_delta_steering_error/8(m_vehicle_total)
  eml_delta_steering_error/1(delta_steeringwheeltotal) -> Out1/1
  In7/1 -> eml_delta_steering_error/7(CorneringStiffness_Tyres_Rear)
  In6/1 -> eml_delta_steering_error/6(CorneringStiffness_Tyres_Front)
  In5/1 -> eml_delta_steering_error/5(yawrate_vehicle)
  In4/1 -> eml_delta_steering_error/4(v_y_vehicle)
  In1/1 -> eml_delta_steering_error/1(v_x_vehicle)

== system tcp_ip/Roewe_550_S_Sedan_1/PathFollower_Preview_1/LateralController/SteeringWheelAngle ==
  Angle_Steering[rad] : Inport
  i_Steering[] : Inport  Port=2
  Angle_SteeringWheel_Last[deg] : Inport  Port=3
  LatCtrl1_Enable[0Off|1On] : Inport  Port=4
  Angle_Max_SteeringWheel[deg]1 : Constant  Value=Angle_Max_SteeringWheel  SampleTime=CSSampleTime
  Const_t_PT1_LatCtrl[s] : Constant  Value=DelayTime  SampleTime=CSSampleTime
  FirstOrderDynamics : Subsystem  mask(First Order Dynamics){}
      mask Display:
      | port_label('input',1,'In')
      | port_label('input',2,'T')
      | port_label('input',3,'Reset')
      | port_label('input',4,'x0')
      | 
      | plot([0.4 0.95], [0.1 0.1]);
      | plot([0.4 0.4], [0.1 0.95]);
      | plot(0.4 + 0.5*[0:0.1:1],0.8- 0.7 * exp(-5*[0:0.1:1]));
  Gain : Gain  SaturateOnIntegerOverflow=on  OutDataTypeStr=Inherit: Same as input  ParamDataTypeStr=Inherit: Same as input
  Product : Product  SaturateOnIntegerOverflow=on  OutDataTypeStr=Inherit: Same as first input
  Rate Limiter : RateLimiter  RisingSlewLimit=MaxSteeringRate  FallingSlewLimit=-MaxSteeringRate  SampleTimeMode=inherited
  Sat_Total : Subsystem
      mask Display:
      | plot([0.25 0.4 0.6 0.75],[0.2 0.2 0.8 0.8])
      | port_label('input',2,'Lim')
      | port_label('output',2,'Info')
  Terminator1 : Terminator
  rad2deg : Gain  Gain=180/pi  SaturateOnIntegerOverflow=on  OutDataTypeStr=Inherit: Same as input  ParamDataTypeStr=Inherit: Same as input
  Angle_SteeringWheel[deg] : Outport  VectorParamsAs1DForOutWhenUnconnected=off
  wires:
  Rate Limiter/1 -> FirstOrderDynamics/1(In)
  Gain/1 -> FirstOrderDynamics/3(Reset)
  Angle_SteeringWheel_Last[deg]/1 -> FirstOrderDynamics/4(x0)
  LatCtrl1_Enable[0Off|1On]/1 -> Gain/1
  Const_t_PT1_LatCtrl[s]/1 -> FirstOrderDynamics/2(TimeConstant[s])
  Sat_Total/2(Sat_Info) -> Terminator1/1
  Angle_Steering[rad]/1 -> rad2deg/1
  i_Steering[]/1 -> Product/2
  rad2deg/1 -> Product/1
  Product/1 -> Sat_Total/1(In)
  Sat_Total/1(Sat_Total) -> Rate Limiter/1
  FirstOrderDynamics/1(Out) -> Angle_SteeringWheel[deg]/1
  Angle_Max_SteeringWheel[deg]1/1 -> Sat_Total/2(Sat_Limit)

== system tcp_ip/Roewe_550_S_Sedan_1/PathFollower_Preview_1/LateralController/s_Preview_LatCtrl ==
  v_x_Vehicle[m|s] : Inport
  v_x_Vehicle_Min[m|s] : Inport  Port=2
  t_Preview_LatCtrl[s] : Inport  Port=3
  Max : MinMax  Function=max  Inputs=2  InputSameDT=on  SaturateOnIntegerOverflow=on
  Prod_s_Min : Product  SaturateOnIntegerOverflow=on  OutDataTypeStr=Inherit: Same as first input
  Product : Product  SaturateOnIntegerOverflow=on  OutDataTypeStr=Inherit: Same as first input
  s_Preview_LatCtrl[m] : Outport  VectorParamsAs1DForOutWhenUnconnected=off
  wires:
  Max/1 -> s_Preview_LatCtrl[m]/1
  Prod_s_Min/1 -> Max/2
  v_x_Vehicle_Min[m|s]/1 -> Prod_s_Min/2
  t_Preview_LatCtrl[s]/1 -> Prod_s_Min/1, Product/2
  Product/1 -> Max/1
  v_x_Vehicle[m|s]/1 -> Product/1

== system tcp_ip/Roewe_550_S_Sedan_1/PathFollower_Preview_1/LongitudinalController/Check_Initial_Velocity ==
  " v_actual_[m|s]" : Inport
  Initial_Velocity_[m|s] : Inport  Port=2
  > eps : simulink/Logic and Bit Operations/Compare To Constant  relop=>  const=0.1  OutDataTypeStr=boolean
  Abs : Abs
  Assertion : Assertion  AssertionFailFcn=warningInitialVelocity(PathFollowerBlockPath);  StopWhenAssertionFail=off
  Constant : Constant  Value=false
  First ? : Memory  InitialCondition=1
  Logical Operator : Logic  AllPortsSameDT=off  OutDataTypeStr=boolean
  Logical Operator1 : Logic  Operator=NOT  AllPortsSameDT=off  OutDataTypeStr=boolean
  Sum : Sum  Inputs=+-
  wires:
  Logical Operator1/1 -> Assertion/1
  Logical Operator/1 -> Logical Operator1/1
  Constant/1 -> First ?/1
  First ?/1 -> Logical Operator/2
  > eps/1 -> Logical Operator/1
  Sum/1 -> Abs/1
  Abs/1 -> > eps/1
  Initial_Velocity_[m|s]/1 -> Sum/2
  " v_actual_[m|s]"/1 -> Sum/1

== system tcp_ip/Roewe_550_S_Sedan_1/PathFollower_Preview_1/LongitudinalController/If Desired Velocity = 0 ==
  In1 : Inport
  Action Port : ActionPort  InitializeStates=reset  PropagateVarSize=During execution  ActionPortLabel=if(u1 == 0)
  constant : Constant  Value=0
  constant1 : Constant  Value=150
  throttle [%] : Outport  InitialOutput=[0]  VectorParamsAs1DForOutWhenUnconnected=off
  brake pressure [bar] : Outport  Port=2  InitialOutput=[150]  VectorParamsAs1DForOutWhenUnconnected=off
  Auto_GearShift : Outport  Port=3  VectorParamsAs1DForOutWhenUnconnected=off
  wires:
  In1/1 -> Auto_GearShift/1
  constant/1 -> throttle [%]/1
  constant1/1 -> brake pressure [bar]/1
